simulink model "WindPlantActivePowerController_Final"  (R2026b)
settings: Solver=ode15s  StopTime=3600
libraries: nesl_utility x6, ee_lib x4, fl_lib x1, eeRmsMeasurement x1
settings Model: Creator=usama  LastModifiedBy=usama
settings DataIOCC: LoggingFileName=C:\Users\usama\Desktop\Matlab Project\GermanWindCurtailmentController\results\Outputs\WindPlant_60min_Final.mat  LoggingToFile=on
settings SimscapeCC: SimscapeNominalValues="[{\"value\":\"1\",\"unit\":\"A\"},{\"value\":\"1\",\"unit\":\"bar\"},{\"value\":\"1\",\"unit\":\"cm^2\"},{\"value\":\"1\",\"unit\":\"cm^3/s\"},{\"value\":\"1\",\"unit\":\"kJ/kg\"},{\"value\":\"1\",\"unit\":\"kW\"},{\"value\":\"1\",\"unit\":\"l\"},{\"value\":\"1\",\"unit\":\"N\"},{\"value\":\"1\",\"unit\":\"N*m\"},{\"value\":\"1\",\"unit\":\"V\"},{\"value\":\"0.001\",\"unit\":\"Wb\"}]"  SimscapeUseEnergyAccounting=off

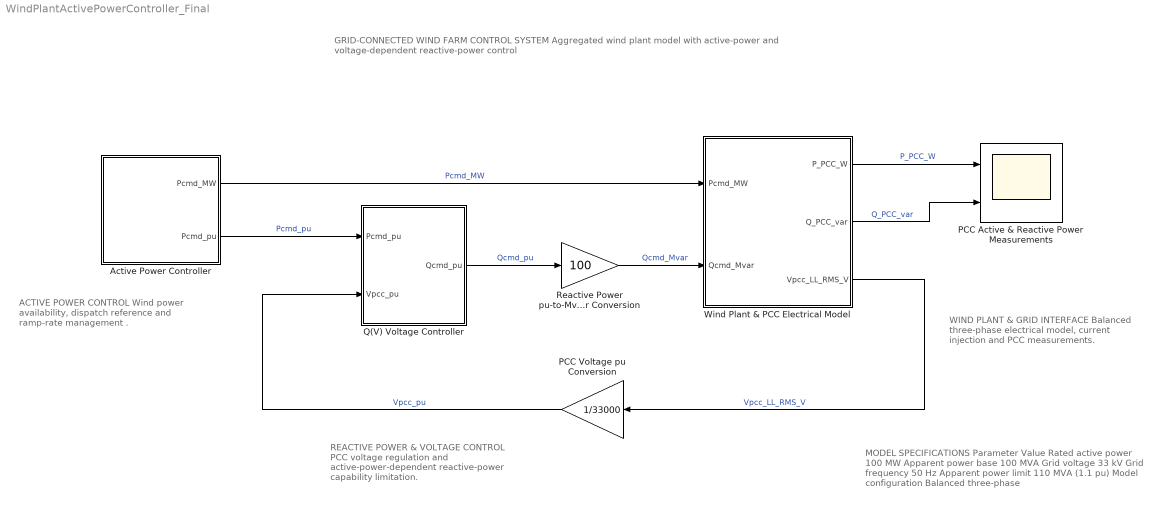
== system WindPlantActivePowerController_Final ==
  note: MODEL SPECIFICATIONS
      |
      | Parameter
      | Value
      |
      | Rated active power
      | 100 MW
      |
      | Apparent power base
      | 100 MVA
      |
      | Grid voltage
      | 33 kV
      |
      | Grid frequency
      | 50 Hz
      |
      | Apparent power limit
      | 110 MVA (1.1 pu)
      |
      | Model configuration
      | Balanced three-phase
  note: ACTIVE POWER CONTROL
      | Wind power availability, dispatch reference and ramp-rate management .
  note: GRID-CONNECTED WIND FARM CONTROL SYSTEM
      |
      | Aggregated wind plant model with active-power and voltage-dependent reactive-power control
  note: REACTIVE POWER & VOLTAGE CONTROL
      | PCC voltage regulation and active-power-dependent reactive-power capability limitation.
  note: WIND PLANT & GRID INTERFACE
      | Balanced three-phase electrical model, current injection and PCC measurements.
  Active Power Controller : Subsystem
  PCC Active & Reactive Power Measurements : Scope  NumInputPorts=2
      settings: ActiveDisplayYMinimum=1.0679699315930868E+6  ActiveDisplayYMaximum=2.2399433473577756E+6  DataLoggingMaxPoints=20000  DataLoggingDecimation=1000  DataLoggingVariableName=ScopeData10
  PCC Voltage pu Conversion : Gain  Gain=1/33000
  Q(V) Voltage Controller : Subsystem
  Reactive Power pu-to-Mvar Conversion : Gain  Gain=100
  Wind Plant & PCC Electrical Model : Subsystem
  wires:
  Q(V) Voltage Controller/1(Qcmd_pu) -> Reactive Power pu-to-Mvar Conversion/1  "Qcmd_pu"
  Wind Plant & PCC Electrical Model/2(Q_PCC_var) -> PCC Active & Reactive Power Measurements/2  "Q_PCC_var"
  Wind Plant & PCC Electrical Model/1("\tP_PCC_W") -> PCC Active & Reactive Power Measurements/1  "P_PCC_W"
  Wind Plant & PCC Electrical Model/3(Vpcc_LL_RMS_V) -> PCC Voltage pu Conversion/1  "Vpcc_LL_RMS_V"
  PCC Voltage pu Conversion/1 -> Q(V) Voltage Controller/2(Vpcc_pu)  "Vpcc_pu"
  Reactive Power pu-to-Mvar Conversion/1 -> Wind Plant & PCC Electrical Model/2(Qcmd_Mvar)  "Qcmd_Mvar"
  Active Power Controller/1(Pcmd_MW) -> Wind Plant & PCC Electrical Model/1(Pcmd_MW)  "Pcmd_MW"
  Active Power Controller/2(Pcmd_pu) -> Q(V) Voltage Controller/1(Pcmd_pu)  "Pcmd_pu"

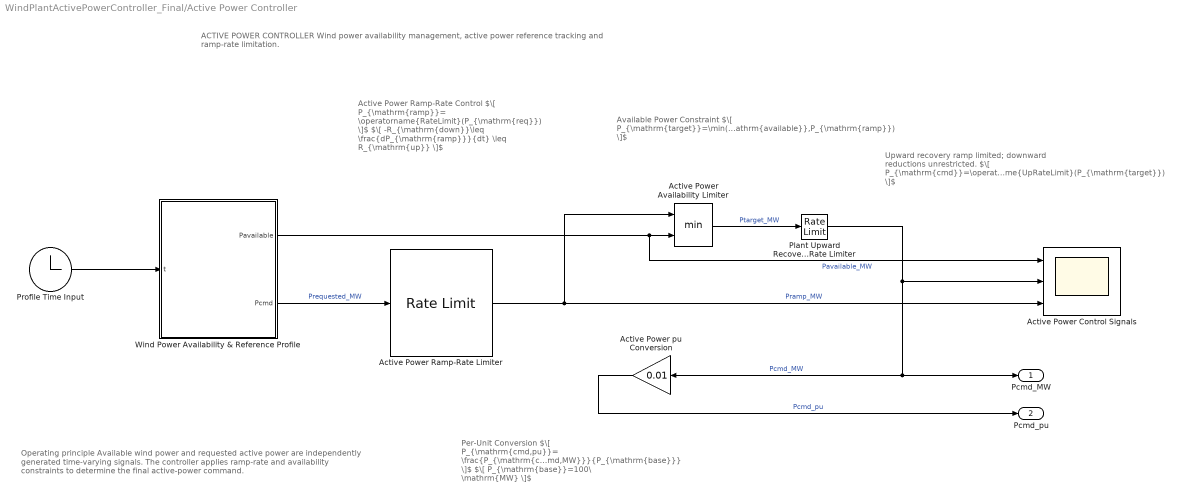
== system WindPlantActivePowerController_Final/Active Power Controller ==
  note: Operating principle
      | Available wind power and requested active power are independently generated time-varying signals. The controller applies ramp-rate and availability constraints to determine the final active-power command.
  note: Available Power Constraint
      |
      | $\[ P_{\mathrm{target}}=\min(P_{\mathrm{available}},P_{\mathrm{ramp}}) \]$
  note: Active Power Ramp-Rate Control
      |
      | $\[ P_{\mathrm{ramp}}= \operatorname{RateLimit}(P_{\mathrm{req}}) \]$
      |
      | $\[ -R_{\mathrm{down}}\leq \frac{dP_{\mathrm{ramp}}}{dt} \leq R_{\mathrm{up}} \]$
  note: ACTIVE POWER CONTROLLER
      | Wind power availability management, active power reference tracking and ramp-rate limitation.
  note: Per-Unit Conversion
      |
      | $\[ P_{\mathrm{cmd,pu}}= \frac{P_{\mathrm{cmd,MW}}}{P_{\mathrm{base}}} \]$
      |
      | $\[ P_{\mathrm{base}}=100\ \mathrm{MW} \]$
  note: Upward recovery ramp limited; downward reductions unrestricted.
      |
      | $\[ P_{\mathrm{cmd}}=\operatorname{UpRateLimit}(P_{\mathrm{target}}) \]$
  Active Power Availability Limiter : MinMax  Inputs=2
  Active Power pu Conversion : Gain  Gain=0.01
  Active Power Ramp-Rate Limiter : RateLimiter  RisingSlewLimit=1/6  FallingSlewLimit=-1/6  SampleTimeMode=inherited  InitialCondition=80
  Active Power Control Signals : Scope  NumInputPorts=3
      settings: ActiveDisplayYMinimum=56.25  ActiveDisplayYMaximum=93.75  DataLoggingMaxPoints=20000  DataLoggingDecimation=1000
  Plant Upward Recovery Rate Limiter : RateLimiter  RisingSlewLimit=1/6  FallingSlewLimit=-inf  SampleTimeMode=inherited  InitialCondition=80
  Profile Time Input : Clock
  Wind Power Availability & Reference Profile : MATLAB Function  TreatAsAtomicUnit=on
  Pcmd_MW : Outport
  Pcmd_pu : Outport  Port=2
  wires:
  Wind Power Availability & Reference Profile/2(Pcmd) -> Active Power Ramp-Rate Limiter/1  "Prequested_MW"
  Active Power Availability Limiter/1 -> Plant Upward Recovery Rate Limiter/1  "Ptarget_MW"
  Profile Time Input/1 -> Wind Power Availability & Reference Profile/1(t)
  Active Power Ramp-Rate Limiter/1 -> Active Power Availability Limiter/1, Active Power Control Signals/3  "Pramp_MW"
  Wind Power Availability & Reference Profile/1(Pavailable) -> Active Power Availability Limiter/2, Active Power Control Signals/1  "Pavailable_MW"
  Active Power pu Conversion/1 -> Pcmd_pu/1  "Pcmd_pu"
  Plant Upward Recovery Rate Limiter/1 -> Active Power pu Conversion/1, Pcmd_MW/1, Active Power Control Signals/2  "Pcmd_MW"

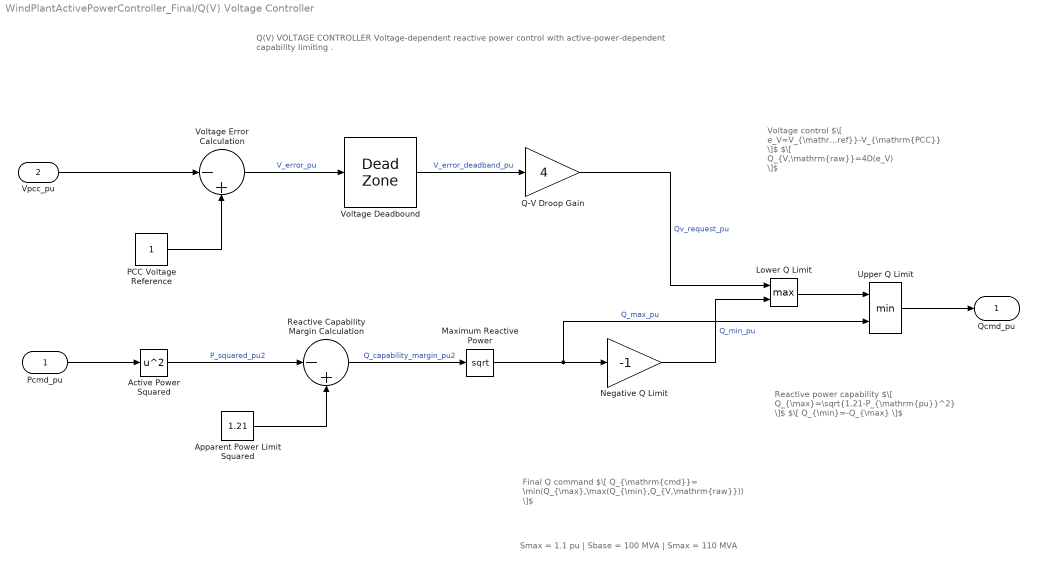
== system WindPlantActivePowerController_Final/Q(V) Voltage Controller ==
  note: Smax = 1.1 pu | Sbase = 100 MVA | Smax = 110 MVA
  note: Final Q command
      |
      | $\[ Q_{\mathrm{cmd}}= \min(Q_{\max},\max(Q_{\min},Q_{V,\mathrm{raw}})) \]$
  note: Reactive power capability
      | $\[ Q_{\max}=\sqrt{1.21-P_{\mathrm{pu}}^2} \]$
      |
      | $\[ Q_{\min}=-Q_{\max} \]$
  note: Voltage control
      |
      | $\[ e_V=V_{\mathrm{ref}}-V_{\mathrm{PCC}} \]$
      |
      | $\[ Q_{V,\mathrm{raw}}=4D(e_V) \]$
  note: Q(V) VOLTAGE CONTROLLER
      | Voltage-dependent reactive power control with active-power-dependent capability limiting .
  Pcmd_pu : Inport
  Vpcc_pu : Inport  Port=2
  "\tNegative Q Limit" : Gain  Gain=-1
  Active Power Squared : Math  Operator=square
  Apparent Power Limit Squared : Constant  Value=1.21
  Lower Q Limit : MinMax  Function=max  Inputs=2
  Maximum Reactive Power : Sqrt
  PCC Voltage Reference : Constant
  Q-V Droop Gain : Gain  Gain=4
  Reactive Capability Margin Calculation : Sum  Inputs=|-+
  Upper Q Limit : MinMax  Inputs=2
  Voltage Deadbound : DeadZone  LowerValue=-0.01  UpperValue=0.01
  Voltage Error Calculation : Sum  Inputs=|-+
  Qcmd_pu : Outport
  wires:
  Voltage Error Calculation/1 -> Voltage Deadbound/1  "V_error_pu"
  Voltage Deadbound/1 -> Q-V Droop Gain/1  "V_error_deadband_pu"
  PCC Voltage Reference/1 -> Voltage Error Calculation/2
  Apparent Power Limit Squared/1 -> Reactive Capability Margin Calculation/2
  Active Power Squared/1 -> Reactive Capability Margin Calculation/1  "P_squared_pu2"
  Reactive Capability Margin Calculation/1 -> Maximum Reactive Power/1  "Q_capability_margin_pu2"
  Maximum Reactive Power/1 -> Upper Q Limit/2, "\tNegative Q Limit"/1  "Q_max_pu"
  "\tNegative Q Limit"/1 -> Lower Q Limit/2  "Q_min_pu"
  Q-V Droop Gain/1 -> Lower Q Limit/1  "Qv_request_pu"
  Lower Q Limit/1 -> Upper Q Limit/1
  Vpcc_pu/1 -> Voltage Error Calculation/1
  Pcmd_pu/1 -> Active Power Squared/1
  Upper Q Limit/1 -> Qcmd_pu/1

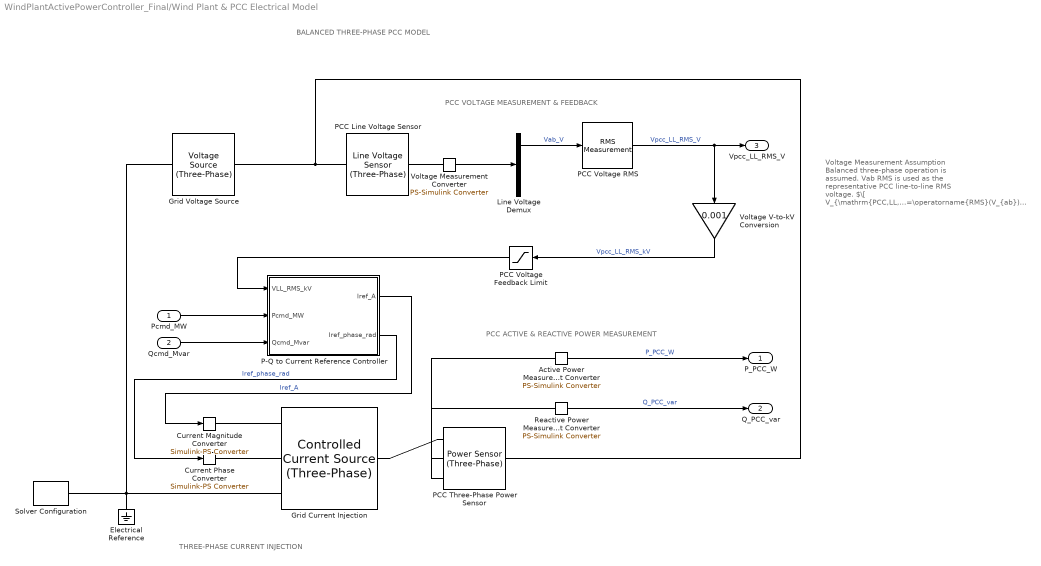
== system WindPlantActivePowerController_Final/Wind Plant & PCC Electrical Model ==
  note: Voltage Measurement Assumption
      |
      | Balanced three-phase operation is assumed. Vab RMS is used as the representative PCC line-to-line RMS voltage.
      |
      | $\[ V_{\mathrm{PCC,LL,RMS}}=\operatorname{RMS}(V_{ab}) \]$
  note: PCC ACTIVE & REACTIVE POWER MEASUREMENT
  note: THREE-PHASE CURRENT INJECTION
  note: PCC VOLTAGE MEASUREMENT & FEEDBACK
  note: BALANCED THREE-PHASE PCC MODEL
  Pcmd_MW : Inport
  Qcmd_Mvar : Inport  Port=2
  "\tCurrent Magnitude Converter" : nesl_utility/Simulink-PS Converter  PhysicalDomain=network_engine_domain  SubClassName=ps_input  LeftPortType=input  RightPortType=output  PseudoPeriodic=off  Frequencies=[]  NoiseDistribution=none  NoiseParameters=[]  Unit=A  AffineConversion=off  FilteringAndDerivatives=filter  SimscapeFilterOrder=1  InputFilterTimeConstant=0.001  UdotUserProvided=0
  "\tVoltage Measurement Converter" : nesl_utility/PS-Simulink Converter  PhysicalDomain=network_engine_domain  SubClassName=ps_output  LeftPortType=input  RightPortType=output  PseudoPeriodic=off  Frequencies=[]  VectorFormat=1-D array  Unit=V  AffineConversion=off
  Active Power Measurement Converter : nesl_utility/PS-Simulink Converter  PhysicalDomain=network_engine_domain  SubClassName=ps_output  LeftPortType=input  RightPortType=output  PseudoPeriodic=off  Frequencies=[]  VectorFormat=1-D array  Unit=W  AffineConversion=off
  Current Phase Converter : nesl_utility/Simulink-PS Converter  PhysicalDomain=network_engine_domain  SubClassName=ps_input  LeftPortType=input  RightPortType=output  PseudoPeriodic=off  Frequencies=[]  NoiseDistribution=none  NoiseParameters=[]  Unit=rad  AffineConversion=off  FilteringAndDerivatives=filter  SimscapeFilterOrder=1  InputFilterTimeConstant=0.001  UdotUserProvided=0
  Electrical Reference : fl_lib/Electrical/Electrical Elements/Electrical Reference
  Grid Current Injection : ee_lib/Sources/Controlled Current Source (Three-Phase)  port_option=ee.enum.threePhasePort.composite  input_option=ee.enum.inputType.singleFreqAC  FRated=50 Hz  G_parasitic=0 1/Ohm
  Grid Voltage Source : ee_lib/Sources/Voltage Source (Three-Phase)  vline_rms=33000 V  shift=0 deg  freq=50 Hz  impedance_option=1  SShortCircuit=3000e6 A*V  XR=10  R=0.01 Ohm  L=3.97e-4 H  harmonic_option=0  harmonic_orders=[5, 7, 11, 13]  harmonic_ratios=[.1, .1, .1, .1]  G_parasitic=0 1/Ohm  I_specify=off  I_priority=None  I=[0, 0, 0] A  I_nominal_specify=off  I_nominal_value=1  I_nominal_unit=A
  Line Voltage Demux : Demux  Outputs=3
  P-Q to Current Reference Controller : Subsystem
  PCC Line Voltage Sensor : ee_lib/Sensors & Transducers/Line Voltage Sensor (Three-Phase)  port_option=ee.enum.threePhasePort.composite
  PCC Three-Phase Power Sensor : ee_lib/Sensors & Transducers/Power Sensor (Three-Phase)  port_option=ee.enum.threePhasePort.composite  load_type=ee.enum.passive.type_balanced.balanced  f0=60 Hz
  PCC Voltage RMS : eeRmsMeasurement/RMS Measurement  LabelModeActiveChoice=Total  F=50  SpecifyHarmonics=off  K=[0 1 2]  InitialRMS=33000  Ts=0
      settings: LibrarySourceBlock=|
      | ee_sl_lib/Measurements/RMS
      | Measurement
  PCC Voltage Feedback Limit : Saturate  UpperLimit=36  LowerLimit=30
  Reactive Power Measurement Converter : nesl_utility/PS-Simulink Converter  PhysicalDomain=network_engine_domain  SubClassName=ps_output  LeftPortType=input  RightPortType=output  PseudoPeriodic=off  Frequencies=[]  VectorFormat=1-D array  Unit=W  AffineConversion=off
  Solver Configuration : nesl_utility/Solver Configuration  PhysicalDomain=network_engine_domain  SubClassName=solver  LeftPortType=input  RightPortType=generic  Tones=[]  Harmonics=[]  SimulateNoise=off  Profile=off  UseLocalSampling=off  EnableSwitchedLinearOptims=on  FrequencyDomain=off  UseCCode=off  RelTol=0.001  AbsTol=0.001  MinStep=1e-09  ToWorkspace=off  RevertToSquareIcSolve=off  NumHomotopyIterations=100  PhasorMode=off  PhasorModeNumHarmonics=1  ConsistencySolver=NEWTON_XTOL_AFTER_FTOL  CanonicalOrdering=CANONICAL  OptimizeIntermediates=OPTIMIZED  MulticoreSolverChoice=BACKWARD_EULER  IndexReductionMethod=DerivativeReplacement  DoDC=off  ResidualTolerance=1e-09  ConsistencyTolSource=GLOBAL  ConsistencyAbsTol=0.001  ConsistencyRelTol=0.001  ConsistencyTolFactor=0.001  UseLocalSolver=off  LocalSolverChoice=NE_BACKWARD_EULER_ADVANCER  ResolveIndetEquations=on  FunctionEvalNumThread=1  LocalSolverSampleTime=0.001  DoFixedCost=off  MaxNonlinIter=3  MaxModeIter=2  ComputeImpulses=off  ImpulseIterations=2  LinearAlgebra=auto  LinearAlgebraNumThread=0  EquationFormulation=NE_TIME_EF  DelaysMemoryBudget=1024  AutomaticFiltering=on  FilteringTimeConstant=0.001  PartitionStorageMethod=AS_NEEDED  PartitionMemoryBudget=1024  PartitionMethod=BALANCED  MultibodyUseLocalSolver=off  MultibodyLocalSolverChoice=ODE1  MultibodyLocalSolverSampleTime=0.001
  Voltage V-to-kV Conversion : Gain  Gain=0.001
  "\tP_PCC_W" : Outport
  Q_PCC_var : Outport  Port=2
  Vpcc_LL_RMS_V : Outport  Port=3
  wires:
  "\tVoltage Measurement Converter"/1 -> Line Voltage Demux/1
  Active Power Measurement Converter/1 -> "\tP_PCC_W"/1  "P_PCC_W"
  Reactive Power Measurement Converter/1 -> Q_PCC_var/1  "Q_PCC_var"
  P-Q to Current Reference Controller/2(Iref_phase_rad) -> Current Phase Converter/1  "Iref_phase_rad"
  PCC Voltage RMS/1 -> Vpcc_LL_RMS_V/1, Voltage V-to-kV Conversion/1  "Vpcc_LL_RMS_V"
  Voltage V-to-kV Conversion/1 -> PCC Voltage Feedback Limit/1  "Vpcc_LL_RMS_kV"
  PCC Voltage Feedback Limit/1 -> P-Q to Current Reference Controller/1(VLL_RMS_kV)
  Pcmd_MW/1 -> P-Q to Current Reference Controller/2(Pcmd_MW)
  Qcmd_Mvar/1 -> P-Q to Current Reference Controller/3(Qcmd_Mvar)
  Line Voltage Demux/1 -> PCC Voltage RMS/1  "Vab_V"
  P-Q to Current Reference Controller/1(Iref_A) -> "\tCurrent Magnitude Converter"/1  "Iref_A"
  connections:
  Electrical Reference/LConn1 -- Grid Voltage Source/LConn1 -- Solver Configuration/RConn1 -- Grid Current Injection/LConn3
  Grid Voltage Source/RConn1 -- PCC Three-Phase Power Sensor/RConn1 -- PCC Line Voltage Sensor/LConn1
  "\tVoltage Measurement Converter"/LConn1 -- PCC Line Voltage Sensor/RConn1
  "\tCurrent Magnitude Converter"/RConn1 -- Grid Current Injection/LConn1
  Current Phase Converter/RConn1 -- Grid Current Injection/LConn2
  PCC Three-Phase Power Sensor/LConn2 -- Active Power Measurement Converter/LConn1
  PCC Three-Phase Power Sensor/LConn3 -- Reactive Power Measurement Converter/LConn1
  Grid Current Injection/RConn1 -- PCC Three-Phase Power Sensor/LConn1

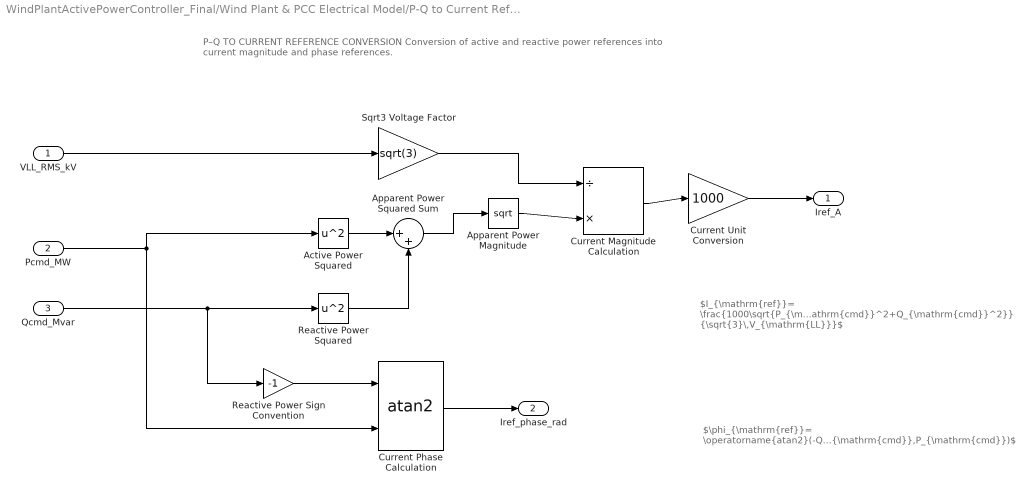
== system WindPlantActivePowerController_Final/Wind Plant & PCC Electrical Model/P-Q to Current Reference Controller ==
  note: $\phi_{\mathrm{ref}}= \operatorname{atan2}(-Q_{\mathrm{cmd}},P_{\mathrm{cmd}})$
  note: $I_{\mathrm{ref}}= \frac{1000\sqrt{P_{\mathrm{cmd}}^2+Q_{\mathrm{cmd}}^2}} {\sqrt{3}\,V_{\mathrm{LL}}}$
  note: P–Q TO CURRENT REFERENCE CONVERSION
      | Conversion of active and reactive power references into current magnitude and phase references.
  VLL_RMS_kV : Inport
  Pcmd_MW : Inport  Port=2
  Qcmd_Mvar : Inport  Port=3
  Active Power Squared : Math  Operator=square
  Apparent Power Magnitude : Sqrt
  Apparent Power Squared Sum : Sum  Inputs=|++
  Current Magnitude Calculation : Product  Inputs=/*
  Current Phase Calculation : Trigonometry  Operator=atan2
  Current Unit Conversion : Gain  Gain=1000
  Reactive Power Squared : Math  Operator=square
  Reactive Power Sign Convention : Gain  Gain=-1
  Sqrt3 Voltage Factor : Gain  Gain=sqrt(3)
  Iref_A : Outport
  Iref_phase_rad : Outport  Port=2
  wires:
  Pcmd_MW/1 -> Current Phase Calculation/2, Active Power Squared/1
  Qcmd_Mvar/1 -> Reactive Power Sign Convention/1, Reactive Power Squared/1
  Active Power Squared/1 -> Apparent Power Squared Sum/1
  Reactive Power Squared/1 -> Apparent Power Squared Sum/2
  Apparent Power Squared Sum/1 -> Apparent Power Magnitude/1
  VLL_RMS_kV/1 -> Sqrt3 Voltage Factor/1
  Current Magnitude Calculation/1 -> Current Unit Conversion/1
  Current Unit Conversion/1 -> Iref_A/1
  Reactive Power Sign Convention/1 -> Current Phase Calculation/1
  Current Phase Calculation/1 -> Iref_phase_rad/1
  Apparent Power Magnitude/1 -> Current Magnitude Calculation/2
  Sqrt3 Voltage Factor/1 -> Current Magnitude Calculation/1

== matlab function WindPlantActivePowerController_Final/Active Power Controller/Wind Power Availability  &  Reference Profile ==
  data: Pavailable output; t input; Pcmd output

function [Pavailable, Pcmd] = fcn(t)
% 100 MW wind farm - 60 minute operating scenario
% t: simulation time in seconds
%
% Pavailable: available wind power (MW)
% Pcmd: requested dispatch power (MW), BEFORE rate limiting
%
% Illustrative engineering test profile, not historical data.

% ---------------------------------------------
% 1. Wind availability profile
% ---------------------------------------------
% Mostly gradual variations with one turbine-group
% outage at 2200 s and gradual recovery afterwards.

time = [ ...
    0  180  360  540  720  900 1080 1200 ...
    1380 1560 1740 1920 2100 2199 2200 2380 ...
    2500 2640 2820 3000 3180 3300 3420 3600];

power = [ ...
    90   91   88   86   84   87   89   88 ...
    85   83   86   89   90   88   58   58 ...
    88   92   90   86   84   76   79   82];

% Piecewise-linear interpolation
if t <= time(1)
    Pavailable = power(1);
elseif t >= time(end)
    Pavailable = power(end);
else
    Pavailable = power(end);

    for k = 1:(length(time)-1)
        if t >= time(k) && t < time(k+1)
            fraction = (t-time(k)) / ...
                (time(k+1)-time(k));

            Pavailable = power(k) + fraction * ...
                (power(k+1)-power(k));
            break;
        end
    end
end

% Small, smooth wind variability outside major events
Pavailable = Pavailable + 0.4*sin(2*pi*t/240);

% Enforce physical 100 MW plant limits
Pavailable = max(0, min(100, Pavailable));

% ---------------------------------------------
% 2. Independent grid dispatch requests
% ---------------------------------------------
if t < 600
    Pcmd = 80;       % Normal export

elseif t < 1200
    Pcmd = 50;       % Curtailment instruction

elseif t < 1700
    Pcmd = 80;       % Curtailment released

elseif t < 2700
    Pcmd = 95;       % High dispatch request

elseif t < 3150
    Pcmd = 65;       % Second curtailment

else
    Pcmd = 90;       % Final recovery
end

end
